simulink model "Planta_e_PI_Exaustao"  (R2026b)
settings: Solver=FixedStepDiscrete  StopTime=160  FixedStep=0.10000000000000001
settings Model: Creator=Guilherme  LastModifiedBy=Guilherme

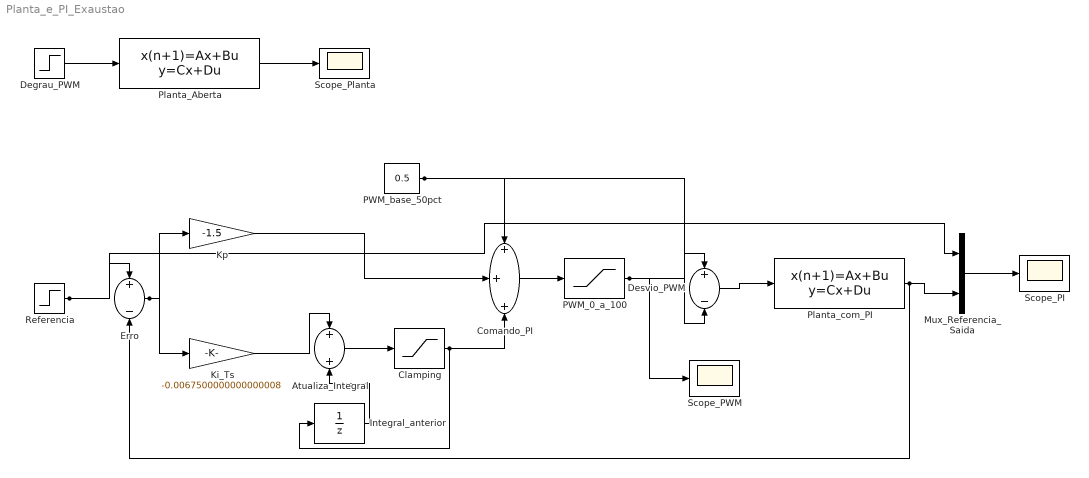
== system Planta_e_PI_Exaustao ==
  Atualiza_Integral : Sum
  Clamping : Saturate
  Comando_PI : Sum  Inputs=+++
  Degrau_PWM : Step  Time=5  FinalValue=0.30  SampleTime=0.1
  Desvio_PWM : Sum  Inputs=+-
  Erro : Sum  Inputs=+-
  Integral_anterior : UnitDelay  SampleTime=0.1
  Ki_Ts : Gain  Gain=-0.0067500000000000008
  Kp : Gain  Gain=-1.5
  Mux_Referencia_Saida : Mux  Inputs=2
  PWM_0_a_100 : Saturate  UpperLimit=1  LowerLimit=0
  PWM_base_50pct : Constant  Value=0.5
  Planta_Aberta : DiscreteStateSpace  A=[0.90822146950116667 -0.04682227211403573 -0.015257268457953671;0.047678963931105225 0.99881150097026661 -0.0003875498462104903;0.00030277331735194555 0.012495010285745003 0.99999837237428624]  B=[0.047678963931105219;0.0012110932694077822;5.0863303555110116e-06]  C=[0 0.10000000000000001 -0.32000000000000001]  D=0  SampleTime=0.10000000000000001
  Planta_com_PI : DiscreteStateSpace  A=[0.90822146950116667 -0.04682227211403573 -0.015257268457953671;0.047678963931105225 0.99881150097026661 -0.0003875498462104903;0.00030277331735194555 0.012495010285745003 0.99999837237428624]  B=[0.047678963931105219;0.0012110932694077822;5.0863303555110116e-06]  C=[0 0.10000000000000001 -0.32000000000000001]  D=0  SampleTime=0.10000000000000001
  Referencia : Step  Time=5  FinalValue=-0.30  SampleTime=0.1
  Scope_PI : Scope
  Scope_PWM : Scope
  Scope_Planta : Scope
  wires:
  Degrau_PWM/1 -> Planta_Aberta/1
  Planta_Aberta/1 -> Scope_Planta/1
  Referencia/1 -> Erro/1, Mux_Referencia_Saida/1
  Erro/1 -> Kp/1, Ki_Ts/1
  Ki_Ts/1 -> Atualiza_Integral/1
  Integral_anterior/1 -> Atualiza_Integral/2
  Atualiza_Integral/1 -> Clamping/1
  Clamping/1 -> Integral_anterior/1, Comando_PI/3
  PWM_base_50pct/1 -> Comando_PI/1, Desvio_PWM/2
  Kp/1 -> Comando_PI/2
  Comando_PI/1 -> PWM_0_a_100/1
  PWM_0_a_100/1 -> Desvio_PWM/1, Scope_PWM/1
  Desvio_PWM/1 -> Planta_com_PI/1
  Planta_com_PI/1 -> Erro/2, Mux_Referencia_Saida/2
  Mux_Referencia_Saida/1 -> Scope_PI/1
